simulink model "tf_zpk"  (R2025b)
settings: Solver=VariableStepAuto  StartTime=0.0  StopTime=10.0  RelTol=1e-3
settings Model: Creator=Shetaab  LastModifiedBy=Shetaab

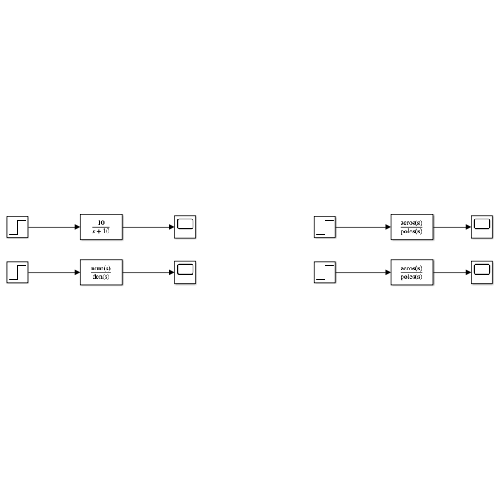
[thumbnail: Simulink's stored preview of the top-level diagram]
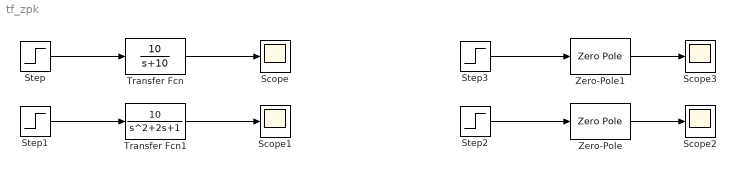
== system tf_zpk ==
  Scope{,1..3} (4 alike) : Scope
      Scope settings: ActiveDisplayYMinimum=-0.12738773145325921  ActiveDisplayYMaximum=1.1225358798296725
      Scope1 settings: ActiveDisplayYMinimum=-0.599288890755207  ActiveDisplayYMaximum=13.904778588550924
      Scope2 settings: ActiveDisplayYMinimum=-2.8451427198823325  ActiveDisplayYMaximum=15.443942751955575  DataLoggingVariableName=ScopeData2
      Scope3 settings: ActiveDisplayYMinimum=-0.11572661621498942  ActiveDisplayYMaximum=0.91111277612710562  DataLoggingVariableName=ScopeData3
  Step{,1..3} (4 alike) : Step  SampleTime=0
  Transfer Fcn : TransferFcn  Numerator=[10]  Denominator=[1 10]
  Transfer Fcn1 : TransferFcn  Numerator=[10]
  Zero-Pole : ZeroPole  Zeros=[]  Poles=[-1 -1]  Gain=[10]
  Zero-Pole1 : ZeroPole  Zeros=[]  Poles=[-10]  Gain=[10]
  wires:
  Step/1 -> Transfer Fcn/1
  Transfer Fcn/1 -> Scope/1
  Transfer Fcn1/1 -> Scope1/1
  Step1/1 -> Transfer Fcn1/1
  Zero-Pole/1 -> Scope2/1
  Step2/1 -> Zero-Pole/1
  Zero-Pole1/1 -> Scope3/1
  Step3/1 -> Zero-Pole1/1
